simulink model "SZ05_ERR_Szinuszos"  (R2026a)
settings: Solver=VariableStepAuto  MaxStep=tau/25
InitFcn:
  | K = 5;
  | tau = 0.125;
  | 
  | y_0 = 2.5;
libraries: MK_SZ x2, simulink_extras x1
settings Model: Creator=Szalay  LastModifiedBy=Szalay

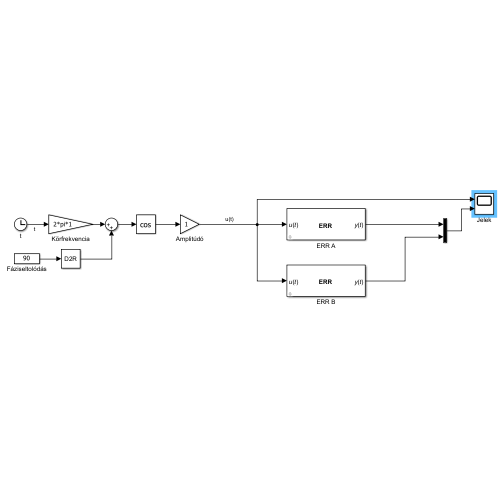
[thumbnail: Simulink's stored preview of the top-level diagram]
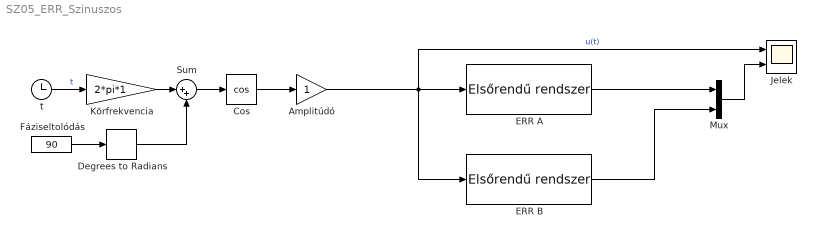
== system SZ05_ERR_Szinuszos ==
  Amplitúdó : Gain
  Cos : Trigonometry  Operator=cos
  Degrees to Radians : simulink_extras/Transformations/Degrees to Radians
  ERR A : MK_SZ/Elsőrendű rendszer  K=1  tau=1  y_0=1.5
  ERR B : MK_SZ/Elsőrendű rendszer  K=1  tau=1  y_0=0
  Fáziseltolódás : Constant  Value=90
  Jelek : Scope  NumInputPorts=2
      settings: ActiveDisplayYMinimum=-0.25049258952841646  ActiveDisplayYMaximum=0.28382633301556504
  Körfrekvencia : Gain  Gain=2*pi*1
  Mux : Mux  Inputs=2
  Sum : Sum  Inputs=|++
  t : Clock
  wires:
  Amplitúdó/1 -> ERR B/1, Jelek/1, ERR A/1  "u(t)"
  Mux/1 -> Jelek/2
  ERR A/1 -> Mux/1
  ERR B/1 -> Mux/2
  t/1 -> Körfrekvencia/1  "t"
  Körfrekvencia/1 -> Sum/1
  Sum/1 -> Cos/1
  Cos/1 -> Amplitúdó/1
  Fáziseltolódás/1 -> Degrees to Radians/1
  Degrees to Radians/1 -> Sum/2
